simulink model "boost_converter"  (R2026b)
settings: Solver=ode23tb
values from neighbouring files (symbols this model uses):
  algo_id = m    [compare_mppt.m]
  C = 470e-6    (= 0.00047)    [boost_params.m]
  Cin = 100e-6    (= 0.0001)    [boost_params.m]
  I0 = (Isc_stc + Ki*(T - T_stc)) / (exp(Voc_T/Vt) - 1)    [compare_mppt.m]    (also in pv_dataset.m; pv_params.m)
  Iph = (Isc_stc + Ki*(T - T_stc)) * (G / G_stc)    [compare_mppt.m]    (also in pv_dataset.m; pv_params.m = 8.21)
  L = 1e-3    (= 0.001)    [boost_params.m]
  R_load = Vout_ref^2 / 200    (= 11.52)    [boost_params.m]
  Rs = 0.221    [compare_mppt.m]    (also in pv_dataset.m; pv_params.m)
  Rsh = 415.405    [compare_mppt.m]    (also in pv_dataset.m; pv_params.m)
  Ts = 5e-3    (= 0.005)    [boost_params.m]
  Vin_nom = 26.3    [boost_params.m]
  Vt = Ns * n * k * T / q    [compare_mppt.m]    (also in pv_dataset.m; pv_params.m = 1.8036190543)
settings Model: Creator=Mark  LastModifiedBy=marklivshits

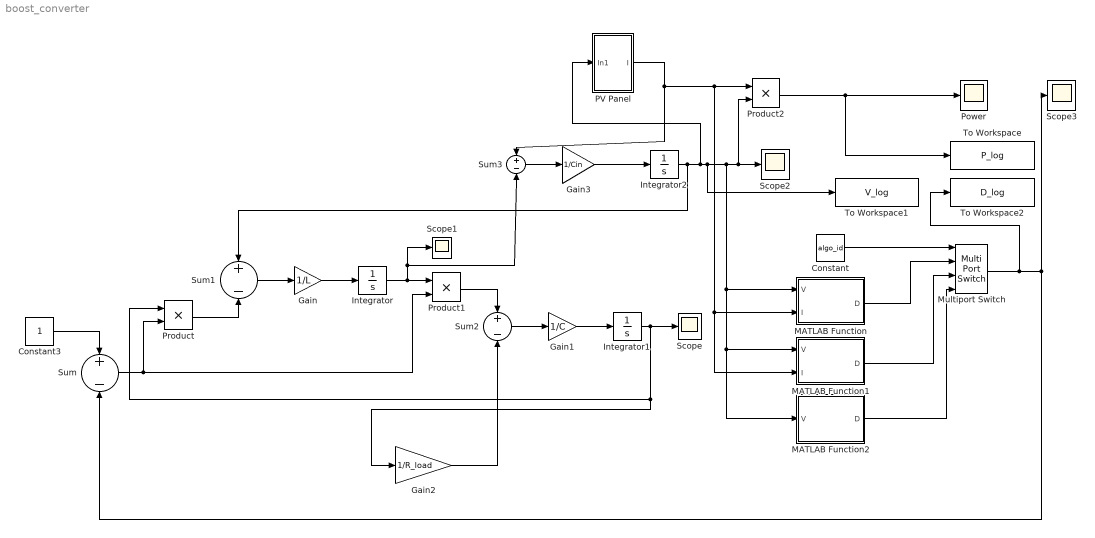
== system boost_converter ==
  Constant : Constant  Value=algo_id
  Constant3 : Constant
  Gain : Gain  Gain=1/L
  Gain1 : Gain  Gain=1/C
  Gain2 : Gain  Gain=1/R_load
  Gain3 : Gain  Gain=1/Cin
  Integrator : Integrator
  Integrator1 : Integrator
  Integrator2 : Integrator  InitialCondition=Vin_nom
  MATLAB Function : MATLAB Function  TreatAsAtomicUnit=on  SystemSampleTime=Ts
  MATLAB Function1 : MATLAB Function  TreatAsAtomicUnit=on  SystemSampleTime=Ts
  MATLAB Function2 : MATLAB Function  TreatAsAtomicUnit=on  SystemSampleTime=Ts
  Multiport Switch : MultiPortSwitch  SaturateOnIntegerOverflow=off  InputSameDT=off
  PV Panel : Subsystem
  Power : Scope
      settings: ActiveDisplayYMinimum=-198.86167926966266  ActiveDisplayYMaximum=253.98221358389856  DataLoggingVariableName=ScopeData3
  Product : Product
  Product1 : Product
  Product2 : Product
  Scope{,1..3} (4 alike) : Scope
      Scope settings: ActiveDisplayYMinimum=28.147743076261676  ActiveDisplayYMaximum=49.686408664941069
      Scope1 settings: ActiveDisplayYMinimum=-1.3230479054962831  ActiveDisplayYMaximum=19.553410987948386
      Scope2 settings: ActiveDisplayYMinimum=25.175620656729318  ActiveDisplayYMaximum=26.755453293578217  DataLoggingVariableName=ScopeData2
      Scope3 settings: ActiveDisplayYMinimum=0.27299999999999985  ActiveDisplayYMaximum=0.47300000000000003  DataLoggingVariableName=ScopeData4
  Sum{,1..3} (4 alike) : Sum  Inputs=+-
  To Workspace : ToWorkspace  VariableName=P_log  SaveFormat=Timeseries  SampleTime=-1
  To Workspace1 : ToWorkspace  VariableName=V_log  SaveFormat=Timeseries  SampleTime=-1
  To Workspace2 : ToWorkspace  VariableName=D_log  SaveFormat=Timeseries  SampleTime=-1
  wires:
  Sum/1 -> Product1/2, Product/2
  Constant3/1 -> Sum/1
  Sum1/1 -> Gain/1
  Product/1 -> Sum1/2
  Gain/1 -> Integrator/1
  Integrator/1 -> Sum3/2, Scope1/1, Product1/1
  Product1/1 -> Sum2/1
  Gain2/1 -> Sum2/2
  Sum2/1 -> Gain1/1
  Gain1/1 -> Integrator1/1
  Integrator1/1 -> Gain2/1, Product/1, Scope/1
  PV Panel/1(I) -> MATLAB Function/2(I), MATLAB Function1/2(I), Product2/1, Sum3/1
  Sum3/1 -> Gain3/1
  Gain3/1 -> Integrator2/1
  Integrator2/1 -> Sum1/1, To Workspace1/1, MATLAB Function/1(V), MATLAB Function1/1(V), MATLAB Function2/1(V), Product2/2, Scope2/1, PV Panel/1(In1)
  Product2/1 -> To Workspace/1, Power/1
  Multiport Switch/1 -> To Workspace2/1, Scope3/1, Sum/2
  Constant/1 -> Multiport Switch/1
  MATLAB Function/1(D) -> Multiport Switch/2
  MATLAB Function1/1(D) -> Multiport Switch/3
  MATLAB Function2/1(D) -> Multiport Switch/4

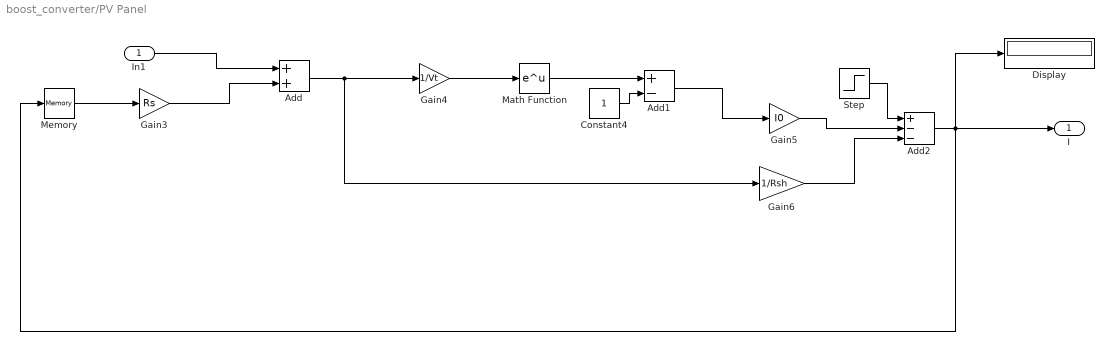
== system boost_converter/PV Panel ==
  In1 : Inport
  Add : Sum
  Add1 : Sum  Inputs=+-
  Add2 : Sum  Inputs=+--
  Constant4 : Constant
  Display : Display
  Gain3 : Gain  Gain=Rs
  Gain4 : Gain  Gain=1/Vt
  Gain5 : Gain  Gain=I0
  Gain6 : Gain  Gain=1/Rsh
  Math Function : Math
  Memory : Memory
  Step : Step  Time=5  InitialValue=Iph  FinalValue=0.6*Iph  SampleTime=0
  I : Outport
  wires:
  Gain5/1 -> Add2/2
  Gain4/1 -> Math Function/1
  Add2/1 -> I/1, Memory/1, Display/1
  Math Function/1 -> Add1/1
  Memory/1 -> Gain3/1
  Add/1 -> Gain4/1, Gain6/1
  Gain3/1 -> Add/2
  Add1/1 -> Gain5/1
  Constant4/1 -> Add1/2
  Gain6/1 -> Add2/3
  In1/1 -> Add/1
  Step/1 -> Add2/1

== matlab function boost_converter/MATLAB Function ==
  data: V input; D output; I input
function D = pno_mppt(V, I)
% Perturb & Observe MPPT
persistent Vprev Pprev Dprev
if isempty(Vprev)
    Vprev = 0;
    Pprev = 0;
    Dprev = 0.45;   % start near operating point
end

dD = 0.001;         % perturbation step
Dmin = 0.05;
Dmax = 0.95;

P = V * I;
dP = P - Pprev;
dV = V - Vprev;

% boost: more D -> lower Vpv, so invert direction
if dP > 0
    if dV > 0
        D = Dprev - dD;
    else
        D = Dprev + dD;
    end
else
    if dV > 0
        D = Dprev + dD;
    else
        D = Dprev - dD;
    end
end

D = min(max(D, Dmin), Dmax);

Vprev = V;
Pprev = P;
Dprev = D;
end

== matlab function boost_converter/MATLAB Function2 ==
  data: V input; D output
function D = cv_mppt(V)
% Constant Voltage MPPT (Vref = 0.8 * Voc_stc)
persistent Dprev
if isempty(Dprev)
    Dprev = 0.45;   % same start
end

Vref = 0.8 * 32.9;  % 26.32 V
Ki   = 0.002;       % integral gain (smooth convergence, no ripple)
Dmin = 0.05;
Dmax = 0.95;

D = Dprev + Ki * (V - Vref);
D = min(max(D, Dmin), Dmax);

Dprev = D;
end

== matlab function boost_converter/MATLAB Function1 ==
  data: V input; D output; I input
function D = inccond_mppt(V, I)
% Incremental Conductance MPPT with relative deadband
persistent Vprev Iprev Dprev
if isempty(Vprev)
    Vprev = 0;
    Iprev = 0;
    Dprev = 0.45;   % same start as P&O
end

dD      = 0.001;    % same step as P&O
Dmin    = 0.05;
Dmax    = 0.95;

eps_V = 1e-3;       % was 1e-4, ignores tiny residual ringing
eps_I   = 1e-4;     % threshold for dI ~ 0
eps_rel = 0.08;     % 8% relative deadband (scales with irradiance)

dV = V - Vprev;
dI = I - Iprev;
D  = Dprev;         % default: hold position at MPP

if abs(V) < 1e-3
    % startup guard against division by zero
    D = Dprev;
elseif abs(dV) < eps_V
    if abs(dI) < eps_I
        % no change -> stay
    elseif dI > 0
        D = Dprev - dD;     % irradiance up -> raise Vpv -> lower D
    else
        D = Dprev + dD;     % irradiance down -> lower Vpv -> raise D
    end
else
    G_inst = I / V;         % instantaneous conductance
    err = (dI / dV) + G_inst;
    if abs(err) <= eps_rel * abs(G_inst)
        % at MPP -> stay (no oscillation)
    elseif err > 0
        D = Dprev - dD;     % left of MPP -> raise Vpv -> lower D
    else
        D = Dprev + dD;     % right of MPP -> lower Vpv -> raise D
    end
end

D = min(max(D, Dmin), Dmax);

Vprev = V;
Iprev = I;
Dprev = D;
end
